simulink model "DCFastCharger"  (R2026b)
settings: Solver=ode23t  StopTime=simulation.simTime  MaxStep=1/(5*inverter.SwitchFrequency)  AbsTol=1e-3
PreLoadFcn:
  | run('DCFastChargerData.mlx');
undefined symbols (not defined in the file or in its folder): battery, inverter, rectifier
libraries: nesl_utility x34, fl_lib x22, ee_lib x14, eePwmGenerator x2, eeTransforms x2, batteryecm_lib x1, eeSinusoidalMeasurement x1, slpidlib x1, eePwmGeneratorThreeLevel x1, eePwmGeneratorTwoLevel x1, simulink_extras x1
(part 3 of 3)

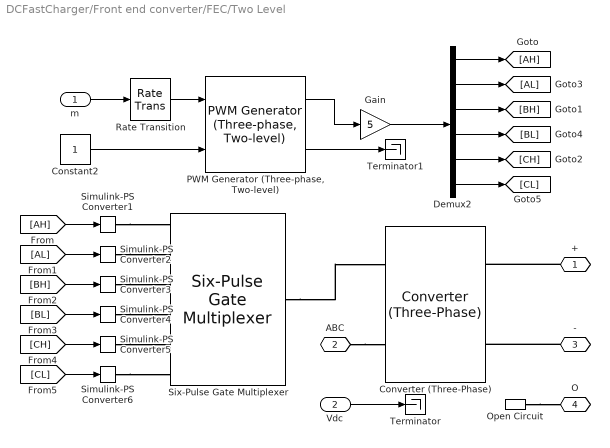
== system DCFastCharger/Front end converter/FEC/Two Level ==
  m : Inport
  Vdc : Inport  Port=2
  Constant2 : Constant
  Converter (Three-Phase) : ee_lib/Semiconductors & Converters/Converters/Converter (Three-Phase)  port_option=ee.enum.threePhasePort.composite  fidelity_option=ee.enum.converters.fidelity.detailed  device_type=ee.enum.converters.switchingdevice.ideal  showThermalPort=false  K=0  Vth=0.5 V  Vgt=1 V  Vgt_off=-1 V  Ih=1 A  Vf=0.8 V  Ron=0.001 Ohm  Rds=0.001 Ohm  Goff=1e-6 1/Ohm  Eon_scalar=22.86e-3 J  Eoff_scalar=17.14e-3 J  Eoff_natural_commutation=10e-3 J  Voff=300 V  Iout_scalar=600 A  onCurrentMeasDelay=0 s  useCurrentFromPreviousCycle=false  useVoltageFromPreviousCycle=false  diode_param=ee.enum.converters.protectiondiode.nodynamics  diode_Vf=0.06 V  diode_Ron=0.001 Ohm  diode_Goff=1e-5 1/Ohm  diode_C=50 nF  diode_iRM=-235 A  diode_iF=300 A  diode_idot=-50 A/us  diode_trr_param=ee.enum.converters.diodetrr.trr_factor  diode_trr_factor=3  diode_trr=15 us  diode_Qrr=1500 s*uA  diode_rec_loss_model=ee.enum.diode.reverseRecoveryModel.fixed  diode_ErecVal=0 J  diode_scaleWithIandV=false  diode_ErecMat=zeros(2, 3) J  diode_TjrecVec=[298.15, 398.15] K  diode_IfrecVec=[.1, 1, 10] A  diode_IrecVal=10 A  diode_VrecVal=10 V  diode_tFilter=1 / 1000 / 100 s  thermal_network_parameterization=ee.enum.thermalNetworkTopology.external  Rth=[.08, .5] K/W  Rth_Cauer=[.08, .1, .5] K/W  Rth_Foster=[.08, .14, .22, .16] K/W  thermal_mass_parameterization=ee.enum.thermalNetwork.timeconstant  thermal_mass=[.01, .5] J/K  thermal_mass_Cauer=[.01, .1, .5] J/K  thermal_mass_Foster=[.001, .005, .05, .5] J/K  thermal_time_constant=[.001, .2] s  thermal_time_constant_Cauer=[.001, .1, .2] s  thermal_time_constant_Foster=[7e-05, .0007, .01, .08] s  thermal_mass_initial_temperatures=[25, 25] degC  thermal_mass_initial_temperatures_Cauer=[25, 25, 25] degC  junction_thermal_mass=0.01 J/K  Tvec_initial_Foster=[25, 25, 25, 25] degC  snubber_type=ee.enum.converters.snubber.exclude  Cs=1e-7 F  Rs=0.1 Ohm  Vce_loss=[0, 150, 300] V
  Demux2 : Demux  Outputs=6
  Gain : Gain  Gain=5
  Open Circuit : fl_lib/Electrical/Electrical Elements/Open Circuit  v_specify=off  v_priority=None  v=0 V  v_nominal_specify=off  v_nominal_value=1  v_nominal_unit=V
  "PWM Generator (Three-phase, Two-level)" : eePwmGeneratorTwoLevel/PWM Generator (Three-phase, Two-level)  PWMMode=Continuous PWM (CPWM)  CPWMMode=SVM: space vector modulation  DPWMMode=60 DPWM: 60 degree discontinuous PWM  fsw=rectifier.SwitchFrequency  Ts=rectifier.VoltageSensorT
  Rate Transition : RateTransition  OutPortSampleTime=rectifier.VoltageSensorT
  Simulink-PS Converter{1..6} (6 alike) : nesl_utility/Simulink-PS Converter  PhysicalDomain=network_engine_domain  SubClassName=ps_input  LeftPortType=input  RightPortType=output  PseudoPeriodic=off  Frequencies=[]  NoiseDistribution=none  NoiseParameters=[]  Unit=1  AffineConversion=off  FilteringAndDerivatives=provide  SimscapeFilterOrder=1  InputFilterTimeConstant=0.001  UdotUserProvided=0
  Six-Pulse Gate Multiplexer : ee_lib/Semiconductors & Converters/Converters/Six-Pulse Gate Multiplexer  port_option=ee.enum.controlport.ps
  Terminator : Terminator
  Terminator1 : Terminator
  + : PMIOPort  Side=Right
  ABC : PMIOPort  Port=2  Side=Left
  - : PMIOPort  Port=3  Side=Right
  O : PMIOPort  Port=4  Side=Right
  wires:
  [AH] -> Simulink-PS Converter1/1
  [CL] -> Simulink-PS Converter6/1
  [AL] -> Simulink-PS Converter2/1
  [BL] -> Simulink-PS Converter4/1
  [CH] -> Simulink-PS Converter5/1
  [BH] -> Simulink-PS Converter3/1
  Gain/1 -> Demux2/1
  Rate Transition/1 -> "PWM Generator (Three-phase, Two-level)"/1
  Demux2/2 -> [AL]
  Demux2/1 -> [AH]
  Demux2/5 -> [CH]
  Demux2/3 -> [BH]
  "PWM Generator (Three-phase, Two-level)"/1 -> Gain/1
  Demux2/4 -> [BL]
  Demux2/6 -> [CL]
  Constant2/1 -> "PWM Generator (Three-phase, Two-level)"/2
  m/1 -> Rate Transition/1
  Vdc/1 -> Terminator/1
  "PWM Generator (Three-phase, Two-level)"/2 -> Terminator1/1
  connections:
  ABC/RConn1 -- Converter (Three-Phase)/LConn2
  Simulink-PS Converter1/RConn1 -- Six-Pulse Gate Multiplexer/LConn1
  Simulink-PS Converter2/RConn1 -- Six-Pulse Gate Multiplexer/LConn2
  Simulink-PS Converter3/RConn1 -- Six-Pulse Gate Multiplexer/LConn3
  Simulink-PS Converter4/RConn1 -- Six-Pulse Gate Multiplexer/LConn4
  Simulink-PS Converter5/RConn1 -- Six-Pulse Gate Multiplexer/LConn5
  Simulink-PS Converter6/RConn1 -- Six-Pulse Gate Multiplexer/LConn6
  Six-Pulse Gate Multiplexer/RConn1 -- Converter (Three-Phase)/LConn1
  +/RConn1 -- Converter (Three-Phase)/RConn1
  -/RConn1 -- Converter (Three-Phase)/RConn2
  Open Circuit/LConn1 -- O/RConn1

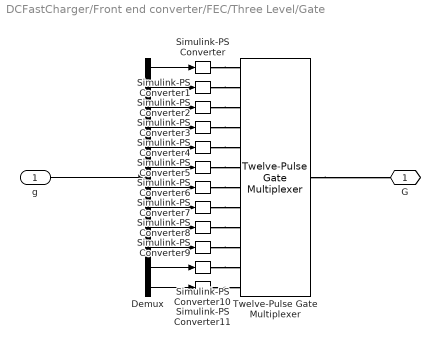
== system DCFastCharger/Front end converter/FEC/Three Level/Gate ==
  g : Inport
  Demux : Demux  Outputs=12
  Simulink-PS Converter{,1..11} (12 alike) : nesl_utility/Simulink-PS Converter  PhysicalDomain=network_engine_domain  SubClassName=ps_input  LeftPortType=input  RightPortType=output  PseudoPeriodic=off  Frequencies=[]  NoiseDistribution=none  NoiseParameters=[]  Unit=1  AffineConversion=off  FilteringAndDerivatives=zero  SimscapeFilterOrder=1  InputFilterTimeConstant=0.001  UdotUserProvided=1
  Twelve-Pulse Gate Multiplexer : ee_lib/Semiconductors & Converters/Converters/Twelve-Pulse Gate Multiplexer  port_option=ee.enum.controlport.ps
  G : PMIOPort  Side=Right
  wires:
  g/1 -> Demux/1
  Demux/5 -> Simulink-PS Converter4/1
  Demux/10 -> Simulink-PS Converter9/1
  Demux/2 -> Simulink-PS Converter1/1
  Demux/9 -> Simulink-PS Converter8/1
  Demux/12 -> Simulink-PS Converter11/1
  Demux/3 -> Simulink-PS Converter2/1
  Demux/7 -> Simulink-PS Converter6/1
  Demux/6 -> Simulink-PS Converter5/1
  Demux/4 -> Simulink-PS Converter3/1
  Demux/1 -> Simulink-PS Converter/1
  Demux/11 -> Simulink-PS Converter10/1
  Demux/8 -> Simulink-PS Converter7/1
  connections:
  Simulink-PS Converter10/RConn1 -- Twelve-Pulse Gate Multiplexer/LConn11
  Simulink-PS Converter8/RConn1 -- Twelve-Pulse Gate Multiplexer/LConn9
  Simulink-PS Converter/RConn1 -- Twelve-Pulse Gate Multiplexer/LConn1
  Simulink-PS Converter11/RConn1 -- Twelve-Pulse Gate Multiplexer/LConn12
  Simulink-PS Converter3/RConn1 -- Twelve-Pulse Gate Multiplexer/LConn4
  Simulink-PS Converter2/RConn1 -- Twelve-Pulse Gate Multiplexer/LConn3
  Simulink-PS Converter4/RConn1 -- Twelve-Pulse Gate Multiplexer/LConn5
  Simulink-PS Converter1/RConn1 -- Twelve-Pulse Gate Multiplexer/LConn2
  Twelve-Pulse Gate Multiplexer/RConn1 -- G/RConn1
  Simulink-PS Converter5/RConn1 -- Twelve-Pulse Gate Multiplexer/LConn6
  Simulink-PS Converter9/RConn1 -- Twelve-Pulse Gate Multiplexer/LConn10
  Simulink-PS Converter6/RConn1 -- Twelve-Pulse Gate Multiplexer/LConn7
  Simulink-PS Converter7/RConn1 -- Twelve-Pulse Gate Multiplexer/LConn8

== system DCFastCharger/Front end converter/FEC/Three Level/Sensing voltage Vc1 ==
  PS-Simulink Converter : nesl_utility/PS-Simulink Converter  PhysicalDomain=network_engine_domain  SubClassName=ps_output  LeftPortType=input  RightPortType=output  PseudoPeriodic=off  Frequencies=[]  VectorFormat=1-D array  Unit=1  AffineConversion=off
  Sensor dynamics : TransferFcn  Numerator=rectifier.VoltageSensorG  Denominator=[rectifier.VoltageSensorT 1]
  Vc1 : fl_lib/Electrical/Electrical Sensors/Voltage Sensor
  + : PMIOPort  Side=Left
  - : PMIOPort  Port=2  Side=Right
  Out1 : Outport
  wires:
  PS-Simulink Converter/1 -> Sensor dynamics/1
  Sensor dynamics/1 -> Out1/1
  connections:
  Vc1/RConn2 -- -/RConn1
  Vc1/LConn1 -- +/RConn1
  PS-Simulink Converter/LConn1 -- Vc1/RConn1

== system DCFastCharger/Front end converter/FEC/Three Level/Sensing voltage Vc2 ==
  PS-Simulink Converter : nesl_utility/PS-Simulink Converter  PhysicalDomain=network_engine_domain  SubClassName=ps_output  LeftPortType=input  RightPortType=output  PseudoPeriodic=off  Frequencies=[]  VectorFormat=1-D array  Unit=1  AffineConversion=off
  Sensor dynamics : TransferFcn  Numerator=rectifier.VoltageSensorG  Denominator=[rectifier.VoltageSensorT 1]
  Vc2 : fl_lib/Electrical/Electrical Sensors/Voltage Sensor
  Conn1 : PMIOPort  Side=Left
  Conn3 : PMIOPort  Port=2  Side=Right
  Out1 : Outport
  wires:
  Sensor dynamics/1 -> Out1/1
  PS-Simulink Converter/1 -> Sensor dynamics/1
  connections:
  Vc2/RConn2 -- Conn3/RConn1
  Vc2/LConn1 -- Conn1/RConn1
  PS-Simulink Converter/LConn1 -- Vc2/RConn1
